simulink model "Hinf_linear_sim"  (R2026a)
settings: Solver=VariableStepAuto
InitFcn:
  | seaDir=fileparts(get_param(bdroot,'FileName'));if isfile(fullfile(seaDir,'..','collaudo_simulink.m')),addpath(fullfile(seaDir,'..'));else,addpath(fullfile(seaDir,'..','..','File_di_Funzioni_Progetto-Accorpati'));end;collaudo_simulink(bdroot);
undefined symbols (not defined in the file): Ak1, Ak2, Aplant, Bk1, Bk2, Bplant, Ck1, Ck2, Cplant, Dk1, Dk2, Dplant, x0plant
libraries: cstblocks_lti x1
settings Model: Creator=rebec  LastModifiedBy=rebec

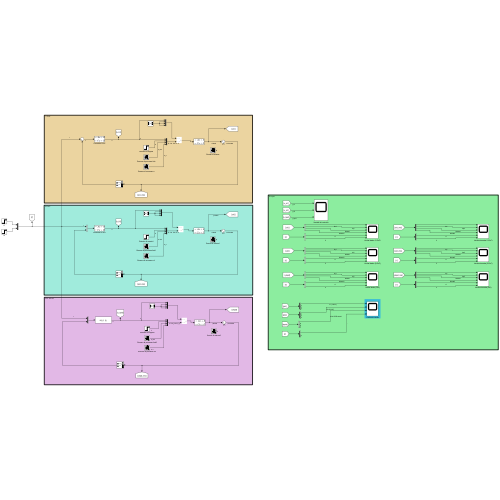
[thumbnail: Simulink's stored preview of the top-level diagram]
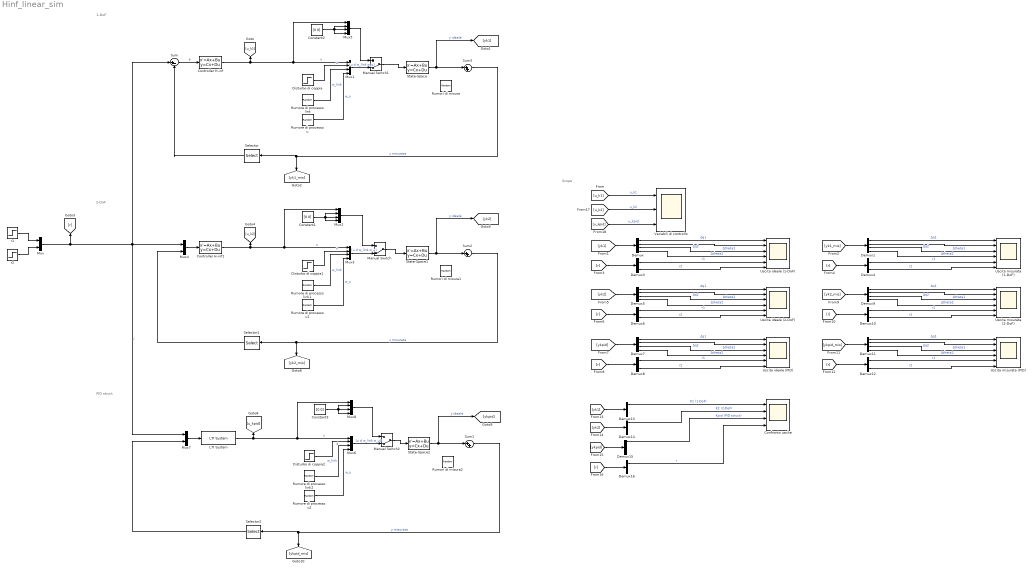
== system Hinf_linear_sim ==
  note: Scope
  note: PID struct
  note: 2-DoF
  note: 1-DoF
  Confronto uscite : Scope  NumInputPorts=4
      settings: Title=Uscite (H-inf)  ActiveDisplayYMinimum=-0.27933944069600969  ActiveDisplayYMaximum=0.21495071578525782  YLabel=y (rad)  DataLoggingVariableName=ScopeData7
  Constant1 : Constant  Value=[0 0]
  Constant2 : Constant  Value=[0 0]
  Constant3 : Constant  Value=[0 0]
  Controller H-inf : StateSpace  A=Ak1  B=Bk1  C=Ck1  D=Dk1  InitialCondition=0
  Controller H-inf1 : StateSpace  A=Ak2  B=Bk2  C=Ck2  D=Dk2  InitialCondition=0
  Demux{,1,5,7,9,11,13..15} (9 alike) : Demux
  Demux{3..4,6,8,10,12,16} (7 alike) : Demux  Outputs=2
  Disturbo di coppia : Step  Time=[1 1]  InitialValue=[0 0]  FinalValue=[0.5 0]  SampleTime=0
  Disturbo di coppia1 : Step  Time=[1 1]  InitialValue=[0 0]  FinalValue=[0.5 0]  SampleTime=0
  Disturbo di coppia2 : Step  Time=[1 1]  InitialValue=[0 0]  FinalValue=[0.5 0]  SampleTime=0
  LTI System : cstblocks_lti/LTI System  sys=Kpid  IC=[]  PadeOrder=0
      settings: LibrarySourceBlock=cstblocks/LTI System
  Manual Switch : ManualSwitch  CurrentSetting=0
  Manual Switch1 : ManualSwitch  CurrentSetting=0
  Manual Switch2 : ManualSwitch  CurrentSetting=0
  Mux : Mux  Inputs=2
  Mux{1..3,5..6,8} (6 alike) : Mux
  Mux4 : Mux  Inputs=2
  Mux7 : Mux  Inputs=2
  Rumore di processo link : RandomNumber  Mean=[0 0]  Variance=[0.01 0.01]  Seed=20260826  SampleTime=0.002
  Rumore di processo link1 : RandomNumber  Mean=[0 0]  Variance=[0.01 0.01]  Seed=20260826  SampleTime=0.002
  Rumore di processo link2 : RandomNumber  Mean=[0 0]  Variance=[0.01 0.01]  Seed=20260826  SampleTime=0.002
  Rumore di processo u : RandomNumber  Mean=[0 0]  Variance=[0.01 0.01]  Seed=20260826  SampleTime=0.002
  Rumore di processo u1 : RandomNumber  Mean=[0 0]  Variance=[0.01 0.01]  Seed=20260826  SampleTime=0.002
  Rumore di processo u2 : RandomNumber  Mean=[0 0]  Variance=[0.01 0.01]  Seed=20260826  SampleTime=0.002
  Rumori di misura : RandomNumber  Mean=[0 0 0 0]  Variance=[(0.05*pi/180)^2 (0.05*pi/180)^2 (0.05*pi/180)^2 (0.05*pi/180)^2]  Seed=20260826  SampleTime=0.002
  Rumori di misura1 : RandomNumber  Mean=[0 0 0 0]  Variance=[(0.05*pi/180)^2 (0.05*pi/180)^2 (0.05*pi/180)^2 (0.05*pi/180)^2]  Seed=20260826  SampleTime=0.002
  Rumori di misura2 : RandomNumber  Mean=[0 0 0 0]  Variance=[(0.05*pi/180)^2 (0.05*pi/180)^2 (0.05*pi/180)^2 (0.05*pi/180)^2]  Seed=20260826  SampleTime=0.002
  Selector : Selector  InputPortWidth=4  IndexOptions=Index vector (dialog)  Indices=[1 2]  OutputSizes=1
  Selector1 : Selector  InputPortWidth=4  IndexOptions=Index vector (dialog)  Indices=[1 2]  OutputSizes=1
  Selector2 : Selector  InputPortWidth=4  IndexOptions=Index vector (dialog)  Indices=[1 2]  OutputSizes=1
  State-Space : StateSpace  A=Aplant  B=Bplant  C=Cplant  D=Dplant  InitialCondition=x0plant
  State-Space1 : StateSpace  A=Aplant  B=Bplant  C=Cplant  D=Dplant  InitialCondition=x0plant
  State-Space2 : StateSpace  A=Aplant  B=Bplant  C=Cplant  D=Dplant  InitialCondition=x0plant
  Sum : Sum  Inputs=|+-
  Sum1 : Sum  Inputs=|++
  Sum2 : Sum  Inputs=|++
  Sum3 : Sum  Inputs=|++
  Uscita ideale (1-DoF) : Scope  NumInputPorts=6
      settings: Title=Uscita ideale (1-DoF)  ActiveDisplayYMinimum=-0.57230265617122578  ActiveDisplayYMaximum=0.50667076569906444  YLabel=y (rad)
  Uscita ideale (2-DoF) : Scope  NumInputPorts=6
      settings: Title=Uscita ideale (2-DoF)  ActiveDisplayYMinimum=-0.30624818665705794  ActiveDisplayYMaximum=0.42404349584753864  YLabel=y (rad)  DataLoggingVariableName=ScopeData3
  Uscita ideale (PID) : Scope  NumInputPorts=6
      settings: Title=Uscita ideale (PID struct)  ActiveDisplayYMinimum=-0.20967372209927659  ActiveDisplayYMaximum=0.28461643438199091  YLabel=y (rad)  DataLoggingVariableName=ScopeData4
  Uscita misurata (1-DoF) : Scope  NumInputPorts=6
      settings: Title=Uscita misurata (1-DoF)  ActiveDisplayYMinimum=-0.57230265617122578  ActiveDisplayYMaximum=0.50667076569906444  YLabel=y_m_i_s (rad)
  Uscita misurata (2-DoF) : Scope  NumInputPorts=6
      settings: Title=Uscita misurata (2-DoF)  ActiveDisplayYMinimum=-0.33288828600734088  ActiveDisplayYMaximum=0.43391798062248577  YLabel=y_m_i_s (rad)  DataLoggingVariableName=ScopeData5
  Uscita misurata (PID) : Scope  NumInputPorts=6
      settings: Title=Uscita misurata (PID struct)  ActiveDisplayYMinimum=-0.20967372209927659  ActiveDisplayYMaximum=0.28461643438199091  YLabel=y_m_i_s (rad)  DataLoggingVariableName=ScopeData6
  Variabili di controllo : Scope  NumInputPorts=3
      settings: ActiveDisplayString=3  Title=PID struct  ActiveDisplayYMinimum=-392.20426405655667  ActiveDisplayYMaximum=429.18075042306987  YLabel=u_k_p_i_d (Nm)  DataLoggingVariableName=ScopeData10
  r1 : Step  FinalValue=5*pi/180  SampleTime=0
  r2 : Step  FinalValue=0  SampleTime=0
  wires:
  r2/1 -> Mux/2
  Sum/1 -> Controller H-inf/1  "e"
  Mux/1 -> Mux4/1, Mux7/1, Sum/1, [r]  "r"
  r1/1 -> Mux/1
  Disturbo di coppia/1 -> Mux1/2  "d"
  Rumore di processo u/1 -> Mux1/4  "w_u"
  Rumore di processo link/1 -> Mux1/3  "w_link"
  State-Space/1 -> [yk1], Sum3/1  "y ideale"
  Sum3/1 -> [yk1_mis], Selector/1  "y misurata"
  Selector/1 -> Sum/2
  State-Space1/1 -> [yk2], Sum2/1  "y ideale"
  Rumore di processo u1/1 -> Mux3/4  "w_u"
  Disturbo di coppia1/1 -> Mux3/2  "d"
  Sum2/1 -> [yk2_mis], Selector1/1  "y misurata"
  Controller H-inf1/1 -> Mux2/1, Mux3/1, [u_k2]  "u"
  State-Space2/1 -> [ykpid], Sum1/1  "y ideale"
  Rumore di processo link1/1 -> Mux3/3  "w_link"
  Sum1/1 -> Selector2/1, [ykpid_mis]  "y misurata"
  Mux7/1 -> LTI System/1
  Mux4/1 -> Controller H-inf1/1
  Selector1/1 -> Mux4/2
  Selector2/1 -> Mux7/2
  Demux/1 -> Uscita ideale (1-DoF)/1  "Δq1"
  Demux/2 -> Uscita ideale (1-DoF)/2  "Δq2"
  [yk1] -> Demux/1
  Mux2/1 -> Manual Switch/1
  Constant1/1 -> Mux2/2, Mux2/4, Mux2/3
  Mux3/1 -> Manual Switch/2  "[u d w_link w_u]"
  Manual Switch/1 -> State-Space1/1
  Constant2/1 -> Mux5/2, Mux5/4, Mux5/3
  Mux5/1 -> Manual Switch1/1
  Controller H-inf/1 -> Mux5/1, Mux1/1, [u_k1]  "u"
  Mux1/1 -> Manual Switch1/2  "[u d w_link w_u]"
  Manual Switch1/1 -> State-Space/1
  Constant3/1 -> Mux8/2, Mux8/4, Mux8/3
  Mux8/1 -> Manual Switch2/1
  LTI System/1 -> Mux8/1, Mux6/1, [u_kpid]  "u"
  Mux6/1 -> Manual Switch2/2  "[u d w_link w_u]"
  Manual Switch2/1 -> State-Space2/1
  Disturbo di coppia2/1 -> Mux6/2  "d"
  Rumore di processo link2/1 -> Mux6/3  "w_link"
  Rumore di processo u2/1 -> Mux6/4  "w_u"
  [r] -> Demux3/1
  Demux3/1 -> Uscita ideale (1-DoF)/5  "r1"
  Demux3/2 -> Uscita ideale (1-DoF)/6  "r2"
  Demux/3 -> Uscita ideale (1-DoF)/3  "Δtheta1"
  Demux/4 -> Uscita ideale (1-DoF)/4  "Δtheta2"
  Demux6/2 -> Uscita ideale (2-DoF)/6  "r2"
  [r] -> Demux6/1
  Demux5/4 -> Uscita ideale (2-DoF)/4  "Δtheta2"
  Demux6/1 -> Uscita ideale (2-DoF)/5  "r1"
  Demux5/1 -> Uscita ideale (2-DoF)/1  "Δq1"
  Demux5/3 -> Uscita ideale (2-DoF)/3  "Δtheta1"
  Demux5/2 -> Uscita ideale (2-DoF)/2  "Δq2"
  [yk2] -> Demux5/1
  [ykpid] -> Demux7/1
  Demux7/2 -> Uscita ideale (PID)/2  "Δq2"
  Demux7/3 -> Uscita ideale (PID)/3  "Δtheta1"
  Demux8/1 -> Uscita ideale (PID)/5  "r1"
  Demux7/4 -> Uscita ideale (PID)/4  "Δtheta2"
  [r] -> Demux8/1
  Demux8/2 -> Uscita ideale (PID)/6  "r2"
  Demux7/1 -> Uscita ideale (PID)/1  "Δq1"
  Demux1/3 -> Uscita misurata (1-DoF)/3  "Δtheta1"
  Demux4/2 -> Uscita misurata (1-DoF)/6  "r2"
  [r] -> Demux4/1
  Demux1/4 -> Uscita misurata (1-DoF)/4  "Δtheta2"
  Demux4/1 -> Uscita misurata (1-DoF)/5  "r1"
  [yk2_mis] -> Demux9/1
  Demux9/3 -> Uscita misurata (2-DoF)/3  "Δtheta1"
  Demux9/2 -> Uscita misurata (2-DoF)/2  "Δq2"
  Demux9/4 -> Uscita misurata (2-DoF)/4  "Δtheta2"
  Demux11/1 -> Uscita misurata (PID)/1  "Δq1"
  Demux11/4 -> Uscita misurata (PID)/4  "Δtheta2"
  Demux11/3 -> Uscita misurata (PID)/3  "Δtheta1"
  Demux12/2 -> Uscita misurata (PID)/6  "r2"
  Demux9/1 -> Uscita misurata (2-DoF)/1  "Δq1"
  [r] -> Demux12/1
  Demux1/1 -> Uscita misurata (1-DoF)/1  "Δq1"
  Demux10/1 -> Uscita misurata (2-DoF)/5  "r1"
  [yk1_mis] -> Demux1/1
  [r] -> Demux10/1
  Demux10/2 -> Uscita misurata (2-DoF)/6  "r2"
  [ykpid_mis] -> Demux11/1
  Demux11/2 -> Uscita misurata (PID)/2  "Δq2"
  Demux1/2 -> Uscita misurata (1-DoF)/2  "Δq2"
  Demux12/1 -> Uscita misurata (PID)/5  "r1"
  [yk1] -> Demux13/1
  Demux13/1 -> Confronto uscite/1  "K1 (1-DoF)"
  [yk2] -> Demux14/1
  Demux14/1 -> Confronto uscite/2  "K2 (2-DoF)"
  [ykpid] -> Demux15/1
  Demux15/1 -> Confronto uscite/3  "Kpid (PID struct)"
  [r] -> Demux16/1
  Demux16/1 -> Confronto uscite/4  "r"
  [u_k1] -> Variabili di controllo/1  "u_k1"
  [u_kpid] -> Variabili di controllo/3  "u_kpid"
  [u_k2] -> Variabili di controllo/2  "u_k2"
